simulink model "BeltStarterGenerator"  (R2024a)
settings: Solver=ode23t  StartTime=0.0  StopTime=0.5  FixedStep=2e-6  RelTol=1e-3  EnableMultiTasking=on
PreLoadFcn:
  | BeltStarterGeneratorData;
undefined symbols (not defined in the file): fswd, Ki_dcdc, Ki_vdc, Kp_dcdc, Kp_vdc, Ld, Lq, p, psim, Tmax, Ts, VDC_VECT
libraries: fl_lib x22, nesl_utility x17, ee_lib x5, eeDiscretePi x3, batteryecm_lib x2, simulink x2, eeTransforms x2, eePmsmCurrentController x1, eePmsmCurrentReferenceGen x1, eePmsmTorqueEstimator x1, eePwmGeneratorTwoLevel x1
(part 2 of 2)

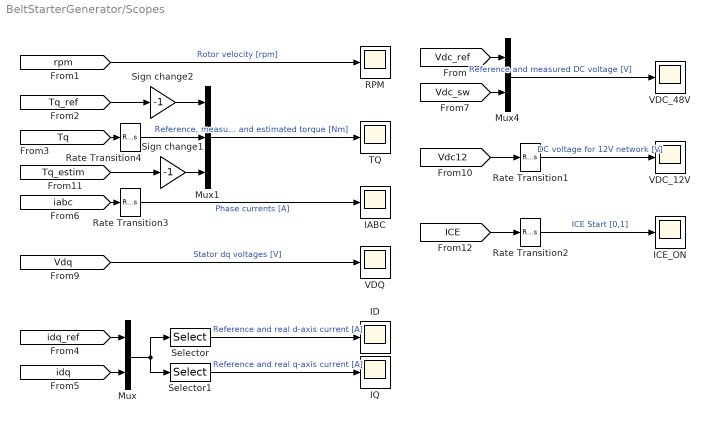
== system BeltStarterGenerator/Scopes ==
  IABC : Scope
  ICE_ON : Scope
  ID : Scope
  IQ : Scope
  Mux : Mux  Inputs=2
  Mux1 : Mux  Inputs=3
  Mux4 : Mux  Inputs=2
  RPM : Scope
  Rate Transition1 : RateTransition  OutPortSampleTime=1e-4
  Rate Transition2 : RateTransition  OutPortSampleTime=1e-4
  Rate Transition3 : RateTransition  OutPortSampleTime=1e-4
  Rate Transition4 : RateTransition
  Selector : Selector  InputPortWidth=4  IndexOptions=Index vector (dialog)  Indices=[1 3]  OutputSizes=1
  Selector1 : Selector  InputPortWidth=4  IndexOptions=Index vector (dialog)  Indices=[2 4]  OutputSizes=1
  Sign change1 : Gain  Gain=-1
  Sign change2 : Gain  Gain=-1
  TQ : Scope
  VDC_12V : Scope
  VDC_48V : Scope
  VDQ : Scope
  wires:
  [rpm] -> RPM/1  "Rotor velocity [rpm]"
  Mux1/1 -> TQ/1  "Reference, measured and estimated torque [Nm]"
  [Tq] -> Rate Transition4/1
  Selector/1 -> ID/1  "Reference and real d-axis current [A]"
  Selector1/1 -> IQ/1  "Reference and real q-axis current [A]"
  [iabc] -> Rate Transition3/1
  [Vdq] -> VDQ/1  "Stator dq voltages [V]"
  Mux4/1 -> VDC_48V/1  "Reference and measured DC voltage [V]"
  [idq_ref] -> Mux/1
  [idq] -> Mux/2
  Mux/1 -> Selector1/1, Selector/1
  [Tq_estim] -> Sign change1/1
  [Vdc_sw] -> Mux4/2
  [Vdc_ref] -> Mux4/1
  Rate Transition3/1 -> IABC/1  "Phase currents [A]"
  [Vdc12] -> Rate Transition1/1
  Rate Transition1/1 -> VDC_12V/1  "DC voltage for 12V network [V]"
  Rate Transition2/1 -> ICE_ON/1  "ICE Start [0,1]"
  [ICE] -> Rate Transition2/1
  [Tq_ref] -> Sign change2/1
  Rate Transition4/1 -> Mux1/2
  Sign change1/1 -> Mux1/3
  Sign change2/1 -> Mux1/1

== system BeltStarterGenerator/Sensor ICE Torque ==
  PS-Simulink Converter3 : nesl_utility/PS-Simulink Converter  PhysicalDomain=network_engine_domain  SubClassName=ps_output  LeftPortType=input  RightPortType=output  PseudoPeriodic=off  Frequencies=[]  VectorFormat=1-D array  Unit=N*m  AffineConversion=off
  Torque Sensor : fl_lib/Mechanical/Mechanical Sensors/Ideal Torque Sensor
  R : PMIOPort  Side=Left
  C : PMIOPort  Port=2  Side=Right
  tag scope: Tq=global
  wires:
  PS-Simulink Converter3/1 -> [Tq]
  connections:
  Torque Sensor/RConn2 -- PS-Simulink Converter3/LConn1
  Torque Sensor/RConn1 -- R/RConn1
  Torque Sensor/LConn1 -- C/RConn1

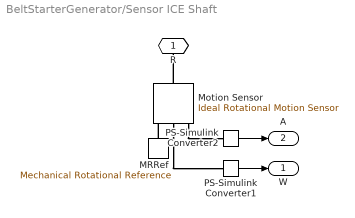
== system BeltStarterGenerator/Sensor ICE Shaft ==
  MRRef : fl_lib/Mechanical/Rotational Elements/Mechanical Rotational Reference
  Motion Sensor : fl_lib/Mechanical/Mechanical Sensors/Ideal Rotational Motion Sensor  reference=foundation.enum.MeasurementReference.difference  acceleration_port=false  velocity_port=true  position_port=true  wrap_angle=simscape.enum.onoff.off  offset=0 deg
  PS-Simulink Converter1 : nesl_utility/PS-Simulink Converter  PhysicalDomain=network_engine_domain  SubClassName=ps_output  LeftPortType=input  RightPortType=output  PseudoPeriodic=off  Frequencies=[]  VectorFormat=1-D array  Unit=rad/s  AffineConversion=off
  PS-Simulink Converter2 : nesl_utility/PS-Simulink Converter  PhysicalDomain=network_engine_domain  SubClassName=ps_output  LeftPortType=input  RightPortType=output  PseudoPeriodic=off  Frequencies=[]  VectorFormat=1-D array  Unit=rad  AffineConversion=off
  R : PMIOPort  Side=Left
  W : Outport  VectorParamsAs1DForOutWhenUnconnected=off
  A : Outport  Port=2  VectorParamsAs1DForOutWhenUnconnected=off
  wires:
  PS-Simulink Converter2/1 -> A/1
  PS-Simulink Converter1/1 -> W/1
  connections:
  Motion Sensor/RConn3 -- PS-Simulink Converter2/LConn1
  MRRef/LConn1 -- Motion Sensor/RConn1
  Motion Sensor/RConn2 -- PS-Simulink Converter1/LConn1
  Motion Sensor/LConn1 -- R/RConn1

== system BeltStarterGenerator/Sensor Phase Currents ==
  Current Sensor : ee_lib/Sensors & Transducers/Current Sensor (Three-Phase)
  PS-Simulink Converter : nesl_utility/PS-Simulink Converter  PhysicalDomain=network_engine_domain  SubClassName=ps_output  LeftPortType=input  RightPortType=output  PseudoPeriodic=off  Frequencies=[]  VectorFormat=1-D array  Unit=A  AffineConversion=off
  1 : PMIOPort  Side=Left
  2 : PMIOPort  Port=2  Side=Right
  tag scope: iabc=global
  wires:
  PS-Simulink Converter/1 -> [iabc]
  connections:
  1/RConn1 -- Current Sensor/LConn1
  Current Sensor/RConn1 -- PS-Simulink Converter/LConn1
  2/RConn1 -- Current Sensor/RConn2

== system BeltStarterGenerator/Sensor V 48V ==
  PS-Simulink Converter5 : nesl_utility/PS-Simulink Converter  PhysicalDomain=network_engine_domain  SubClassName=ps_output  LeftPortType=input  RightPortType=output  PseudoPeriodic=off  Frequencies=[]  VectorFormat=1-D array  Unit=V  AffineConversion=off
  Voltage Sensor : fl_lib/Electrical/Electrical Sensors/Voltage Sensor
  + : PMIOPort  Side=Left
  - : PMIOPort  Port=2  Side=Right
  tag scope: Vdc48=global
  wires:
  PS-Simulink Converter5/1 -> [Vdc48]
  connections:
  -/RConn1 -- Voltage Sensor/RConn2
  PS-Simulink Converter5/LConn1 -- Voltage Sensor/RConn1
  +/RConn1 -- Voltage Sensor/LConn1

== system BeltStarterGenerator/Switch 12V Load ==
  S : Inport
  Simulink-PS Converter2 : nesl_utility/Simulink-PS Converter  PhysicalDomain=network_engine_domain  SubClassName=ps_input  LeftPortType=input  RightPortType=output  PseudoPeriodic=off  Frequencies=[]  NoiseDistribution=none  NoiseParameters=[]  Unit=1  AffineConversion=off  FilteringAndDerivatives=zero  SimscapeFilterOrder=1  InputFilterTimeConstant=0.001  UdotUserProvided=1
  Switch : fl_lib/Electrical/Electrical Elements/Switch  R_closed=0.01 Ohm  G_open=1e-8 1/Ohm  Threshold=0  i_specify=off  i_priority=None  i=0 A  i_nominal_specify=off  i_nominal_value=1  i_nominal_unit=A  v_specify=off  v_priority=None  v=0 V  v_nominal_specify=off  v_nominal_value=1  v_nominal_unit=V
  a : PMIOPort  Side=Left
  b : PMIOPort  Port=2  Side=Right
  wires:
  S/1 -> Simulink-PS Converter2/1
  connections:
  b/RConn1 -- Switch/LConn1
  Simulink-PS Converter2/RConn1 -- Switch/RConn1
  Switch/RConn2 -- a/RConn1

== system BeltStarterGenerator/Switch 48V Load ==
  S : Inport
  Simulink-PS Converter2 : nesl_utility/Simulink-PS Converter  PhysicalDomain=network_engine_domain  SubClassName=ps_input  LeftPortType=input  RightPortType=output  PseudoPeriodic=off  Frequencies=[]  NoiseDistribution=none  NoiseParameters=[]  Unit=1  AffineConversion=off  FilteringAndDerivatives=zero  SimscapeFilterOrder=1  InputFilterTimeConstant=0.001  UdotUserProvided=1
  Switch : fl_lib/Electrical/Electrical Elements/Switch  R_closed=0.01 Ohm  G_open=1e-8 1/Ohm  Threshold=0  i_specify=off  i_priority=None  i=0 A  i_nominal_specify=off  i_nominal_value=1  i_nominal_unit=A  v_specify=off  v_priority=None  v=0 V  v_nominal_specify=off  v_nominal_value=1  v_nominal_unit=V
  a : PMIOPort  Side=Left
  b : PMIOPort  Port=2  Side=Right
  wires:
  S/1 -> Simulink-PS Converter2/1
  connections:
  Switch/RConn2 -- a/RConn1
  Simulink-PS Converter2/RConn1 -- Switch/RConn1
  b/RConn1 -- Switch/LConn1

== system BeltStarterGenerator/DCDC Buck Converter/Sensor V 12V ==
  PS-Simulink Converter5 : nesl_utility/PS-Simulink Converter  PhysicalDomain=network_engine_domain  SubClassName=ps_output  LeftPortType=input  RightPortType=output  PseudoPeriodic=off  Frequencies=[]  VectorFormat=1-D array  Unit=V  AffineConversion=off
  Voltage Sensor : fl_lib/Electrical/Electrical Sensors/Voltage Sensor
  + : PMIOPort  Side=Left
  - : PMIOPort  Port=2  Side=Right
  vdc : Outport  VectorParamsAs1DForOutWhenUnconnected=off
  wires:
  PS-Simulink Converter5/1 -> vdc/1
  connections:
  +/RConn1 -- Voltage Sensor/LConn1
  PS-Simulink Converter5/LConn1 -- Voltage Sensor/RConn1
  -/RConn1 -- Voltage Sensor/RConn2

== system BeltStarterGenerator/DCDC Controller/PWM Generation ==
  DC : Inport
  Counter Limited : simulink/Sources/Counter Limited  uplimit=1/(f*Ts)  tsamp=Ts
  Data Type Conversion1 : DataTypeConversion  SaturateOnIntegerOverflow=off  RndMeth=Floor
  Data Type Conversion2 : DataTypeConversion  SaturateOnIntegerOverflow=off  RndMeth=Floor
  Gain : Gain  Gain=f*Ts
  Relational Operator : RelationalOperator  OutDataTypeStr=boolean  RndMeth=Simplest  InputSameDT=off
  PWM : Outport  VectorParamsAs1DForOutWhenUnconnected=off
  wires:
  Counter Limited/1 -> Data Type Conversion1/1
  Gain/1 -> Relational Operator/2
  Data Type Conversion2/1 -> PWM/1
  Relational Operator/1 -> Data Type Conversion2/1
  DC/1 -> Relational Operator/1
  Data Type Conversion1/1 -> Gain/1

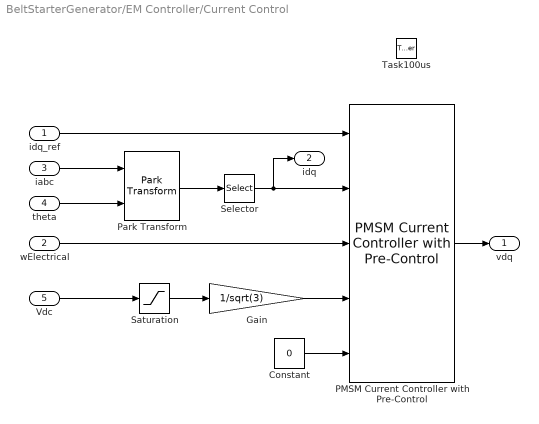
== system BeltStarterGenerator/EM Controller/Current Control ==
  idq_ref : Inport
  wElectrical : Inport  Port=2
  iabc : Inport  Port=3
  theta : Inport  Port=4
  Vdc : Inport  Port=5
  Task100us : TriggerPort  TriggerType=function-call  VariantControl=Variant  PortDimensions=1
  Constant : Constant  Value=0  SampleTime=-1
  Gain : Gain  Gain=1/sqrt(3)
  PMSM Current Controller with Pre-Control : eePmsmCurrentController/PMSM Current Controller with Pre-Control  Kp_id=Kp_id  Ki_id=Ki_id  Kaw_id=1  Kp_iq=Kp_iq  Ki_iq=Ki_iq  Kaw_iq=1  Ts=-1  Tsd=Tsi  AxisPrio=Q-axis  ActZC=on  ActFF=on  idVect=[-200, 0, 200]  iqVect=[-200, 0, 200]  LdMatrix=Ld * ones(3, 3)  LqMatrix=Lq * ones(3, 3)  psimMatrix=psim * ones(3, 3)
  Park Transform : eeTransforms/Park Transform  AxisAlignment=Q-axis  PowerInvariant=off
  Saturation : Saturate  UpperLimit=inf  LowerLimit=VDC_VECT(1)
  Selector : Selector  InputPortWidth=3  IndexOptions=Index vector (dialog)  Indices=[1 2]  OutputSizes=1
  vdq : Outport  VectorParamsAs1DForOutWhenUnconnected=off
  idq : Outport  Port=2  VectorParamsAs1DForOutWhenUnconnected=off
  wires:
  iabc/1 -> Park Transform/1
  Saturation/1 -> Gain/1
  Park Transform/1 -> Selector/1
  theta/1 -> Park Transform/2
  Vdc/1 -> Saturation/1
  idq_ref/1 -> PMSM Current Controller with Pre-Control/1
  PMSM Current Controller with Pre-Control/1 -> vdq/1
  wElectrical/1 -> PMSM Current Controller with Pre-Control/3
  Gain/1 -> PMSM Current Controller with Pre-Control/4
  Constant/1 -> PMSM Current Controller with Pre-Control/5
  Selector/1 -> idq/1, PMSM Current Controller with Pre-Control/2

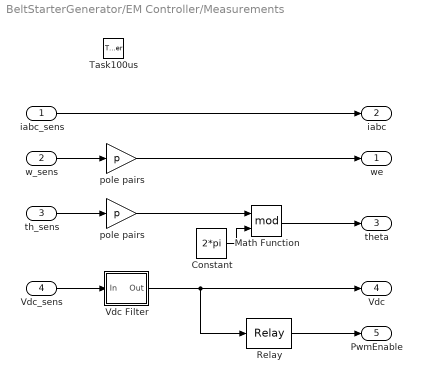
== system BeltStarterGenerator/EM Controller/Measurements ==
  iabc_sens : Inport
  w_sens : Inport  Port=2
  th_sens : Inport  Port=3
  Vdc_sens : Inport  Port=4
  Task100us : TriggerPort  TriggerType=function-call  VariantControl=Variant  PortDimensions=1
  Constant : Constant  Value=2*pi  SampleTime=-1
  Math Function : Math  Operator=mod  SignedPower=on
  Relay : Relay  OnSwitchValue=VDC_VECT(1)  OffSwitchValue=0.5*VDC_VECT(1)
  Vdc Filter : Subsystem  mask(Discrete first-order filter (Low-pass)){T=0.005, Ts=1e-4}
      mask prompts: T "Time constant (s):"; Ts "Sample time (s):"
      mask help: This block implements a discrete low-pass filter. To calculate the coefficients, the block discretises a continuous low-pass filter using the Tustin method.
      mask init:
      | num = [ Ts/(2*T + Ts), Ts/(2*T + Ts)];
      | den = [ 1, -(2*T - Ts)/(2*T + Ts)];
  pole pairs : Gain  Gain=p
  "pole pairs " : Gain  Gain=p
  we : Outport  VectorParamsAs1DForOutWhenUnconnected=off
  iabc : Outport  Port=2  VectorParamsAs1DForOutWhenUnconnected=off
  theta : Outport  Port=3  VectorParamsAs1DForOutWhenUnconnected=off
  Vdc : Outport  Port=4  VectorParamsAs1DForOutWhenUnconnected=off
  PwmEnable : Outport  Port=5  VectorParamsAs1DForOutWhenUnconnected=off
  wires:
  w_sens/1 -> pole pairs/1
  iabc_sens/1 -> iabc/1
  pole pairs/1 -> we/1
  Constant/1 -> Math Function/2
  Math Function/1 -> theta/1
  th_sens/1 -> "pole pairs "/1
  "pole pairs "/1 -> Math Function/1
  Relay/1 -> PwmEnable/1
  Vdc_sens/1 -> Vdc Filter/1(In)
  Vdc Filter/1(Out) -> Relay/1, Vdc/1

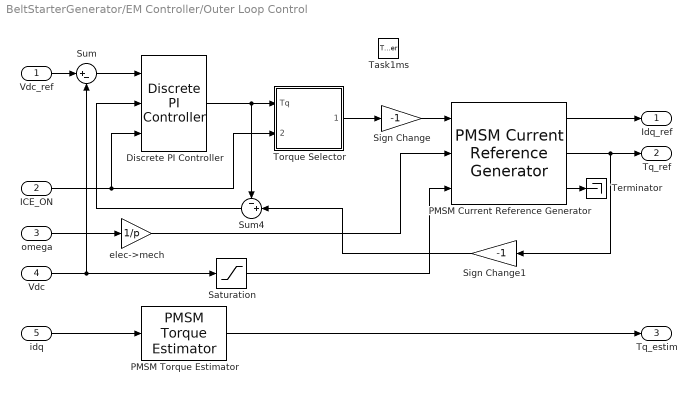
== system BeltStarterGenerator/EM Controller/Outer Loop Control ==
  Vdc_ref : Inport
  ICE_ON : Inport  Port=2
  omega : Inport  Port=3
  Vdc : Inport  Port=4
  idq : Inport  Port=5
  Task1ms : TriggerPort  TriggerType=function-call  VariantControl=Variant  PortDimensions=1
  Discrete PI Controller : eeDiscretePi/Discrete PI Controller  Kp=Kp_vdc  Ki=Ki_vdc  Kaw=1  x0=0  Ts=-1
  PMSM Current Reference Generator : eePmsmCurrentReferenceGen/PMSM Current Reference Generator  Vnom=48  Pmax=Pmax  Tmax=Tmax  Ts=-1  RefType=Lookup-table based  rpmVec=RPM_VECT  TqVec=TQ_VECT  VdcVec=VDC_VECT  PWMMode=SVM: space vector modulation  ModFactor=1  idMatrix=ID_MAP  iqMatrix=IQ_MAP  p=8  psim=0.04  Ld=0.00024  Lq=0.00029  Rs=0.01  RefExpEnable=0
  PMSM Torque Estimator : eePmsmTorqueEstimator/PMSM Torque Estimator  ParamType=Constant parameters  p=p  idVect=[-200, 200]  iqVect=[-200, 200]  LdMatrix=0.0002 * ones(2, 2)  LqMatrix=0.0002 * ones(2, 2)  psimMatrix=0.04 * ones(2, 2)  Ld=Ld  Lq=Lq  psim=psim  Ts=-1
  Saturation : Saturate  UpperLimit=inf  LowerLimit=VDC_VECT(1)
  Sign Change : Gain  Gain=-1
  Sign Change1 : Gain  Gain=-1
  Sum : Sum  Inputs=|+-
  Sum4 : Sum  Inputs=-+|
  Terminator : Terminator
  Torque Selector : Subsystem
  elec->mech : Gain  Gain=1/p
  Idq_ref : Outport  VectorParamsAs1DForOutWhenUnconnected=off
  Tq_ref : Outport  Port=2  VectorParamsAs1DForOutWhenUnconnected=off
  Tq_estim : Outport  Port=3  VectorParamsAs1DForOutWhenUnconnected=off
  wires:
  Sum/1 -> Discrete PI Controller/1
  Vdc_ref/1 -> Sum/1
  Saturation/1 -> PMSM Current Reference Generator/3
  PMSM Torque Estimator/1 -> Tq_estim/1
  omega/1 -> elec->mech/1
  idq/1 -> PMSM Torque Estimator/1
  Discrete PI Controller/1 -> Torque Selector/1(Tq), Sum4/1
  Sum4/1 -> Discrete PI Controller/2
  ICE_ON/1 -> Discrete PI Controller/3, Torque Selector/2(TqSwitch)
  Vdc/1 -> Sum/2, Saturation/1
  elec->mech/1 -> PMSM Current Reference Generator/2
  Torque Selector/1(Tq_ref) -> Sign Change/1
  PMSM Current Reference Generator/1 -> Idq_ref/1
  PMSM Current Reference Generator/2 -> Tq_ref/1, Sign Change1/1
  PMSM Current Reference Generator/3 -> Terminator/1
  Sign Change/1 -> PMSM Current Reference Generator/1
  Sign Change1/1 -> Sum4/2

== system BeltStarterGenerator/EM Controller/Measurements/Vdc Filter ==
  In : Inport
  Discrete Transfer Fcn : DiscreteTransferFcn  Numerator=num  Denominator=den
  Out : Outport  VectorParamsAs1DForOutWhenUnconnected=off
  wires:
  In/1 -> Discrete Transfer Fcn/1
  Discrete Transfer Fcn/1 -> Out/1

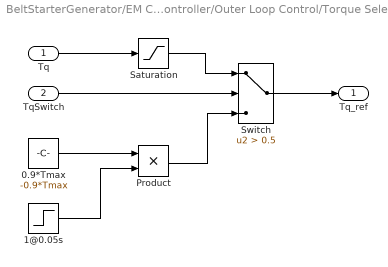
== system BeltStarterGenerator/EM Controller/Outer Loop Control/Torque Selector ==
  Tq : Inport
  TqSwitch : Inport  Port=2
  0.9*Tmax : Constant  Value=-0.9*Tmax  SampleTime=-1
  1@0.05s : Step  Time=0.05
  Product : Product
  Saturation : Saturate  UpperLimit=50  LowerLimit=-10
  Switch : Switch  Criteria=u2 > Threshold  Threshold=0.5  SaturateOnIntegerOverflow=off  InputSameDT=off
  Tq_ref : Outport  VectorParamsAs1DForOutWhenUnconnected=off
  wires:
  Tq/1 -> Saturation/1
  Switch/1 -> Tq_ref/1
  TqSwitch/1 -> Switch/2
  Saturation/1 -> Switch/1
  0.9*Tmax/1 -> Product/1
  1@0.05s/1 -> Product/2
  Product/1 -> Switch/3

== stateflow chart BeltStarterGenerator/EM Controller/Task Scheduler ==
  (default) -> (junction 105) : CLK_50us
  (junction 105) -> (junction 106)
  (junction 106) -> (junction 112) [order 2]
  (junction 106) -> (junction 112) [order 1] : [cnt%%2==0]{Task_100us_1;}
  (junction 112) -> (junction 110) [order 2]
  (junction 112) -> (junction 110) [order 1] : [cnt%%2==0]{Task_100us_2;}
  (junction 110) -> (junction 111) [order 2]
  (junction 110) -> (junction 111) [order 1] : [cnt%%20==0]{Task_1ms_1;}
  (junction 111) -> (junction 107) [order 2]
  (junction 111) -> (junction 108) [order 1] : [1]{cnt++;}
  data: cnt local int32
  events: Task_100us_1 output FUNCTION_CALL_EVENT; Task_100us_2 output FUNCTION_CALL_EVENT; Task_1ms_1 output FUNCTION_CALL_EVENT; CLK_50us input FUNCTION_CALL_EVENT
